simulink model "modelo_data"  (R2025a)
settings: Solver=VariableStepAuto  StartTime=0.0  StopTime=100  RelTol=1e-3
values from neighbouring files (symbols this model uses):
  E0 = E0_values(j)    [data.m]
  T0 = T0_values(i)    [data.m]
settings Model: Creator=cmparedesv  LastModifiedBy=cmparedesv

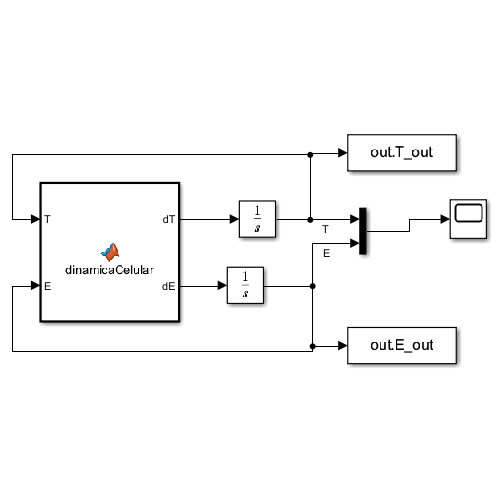
[thumbnail: Simulink's stored preview of the top-level diagram]
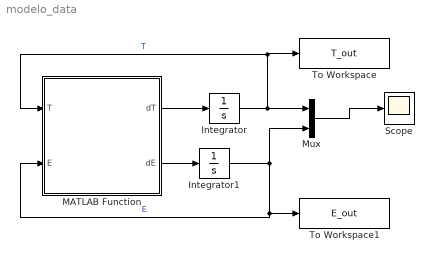
== system modelo_data ==
  Integrator : Integrator  InitialCondition=T0
  Integrator1 : Integrator  InitialCondition=E0
  MATLAB Function : MATLAB Function  TreatAsAtomicUnit=on
  Mux : Mux  Inputs=2
  Scope : Scope
      settings: ActiveDisplayYMinimum=-0.098694986967310355  ActiveDisplayYMaximum=1.3882548827057932
  To Workspace : ToWorkspace  VariableName=T_out  SaveFormat=Timeseries  SampleTime=-1
  To Workspace1 : ToWorkspace  VariableName=E_out  SaveFormat=Timeseries  SampleTime=-1
  wires:
  MATLAB Function/1(dT) -> Integrator/1
  MATLAB Function/2(dE) -> Integrator1/1
  Integrator/1 -> To Workspace/1, MATLAB Function/1(T), Mux/1  "T"
  Integrator1/1 -> Mux/2, To Workspace1/1, MATLAB Function/2(E)  "E"
  Mux/1 -> Scope/1

== matlab function modelo_data/MATLAB Function ==
  data: T input; dT output; E input; dE output
function [dT,dE] = dinamicaCelular(T,E)
r=1.0;
K=1.0;
alpha=0.8;
s=.1;
p = 0.5;
h = 0.3;
delta= .2;
eta = .1

dT = r*T*(1-T/K)-alpha*T*E;
dE = s+p*T*E/(h+T)-delta*E-eta*T*E;
